simulink subsystem "DoubleActingPistonCylinderControlledValves"  (R2025b)
settings: Solver=VariableStepAuto  StartTime=0.0  StopTime=10.0  RelTol=1e-3
libraries: customization_lib x7, nesl_utility x2, fl_lib x1
settings Model: Creator=ndegoede  LastModifiedBy=ndegoede

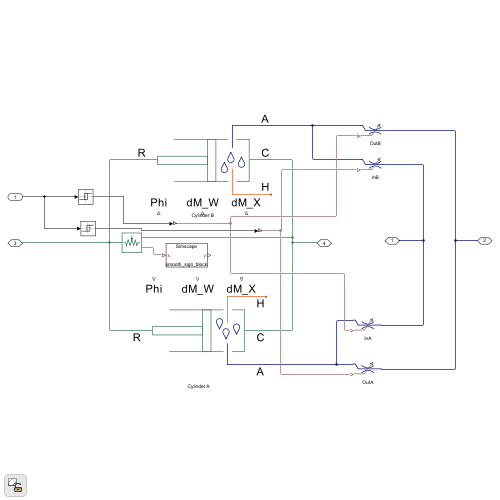
[thumbnail: Simulink's stored preview of the top-level diagram]
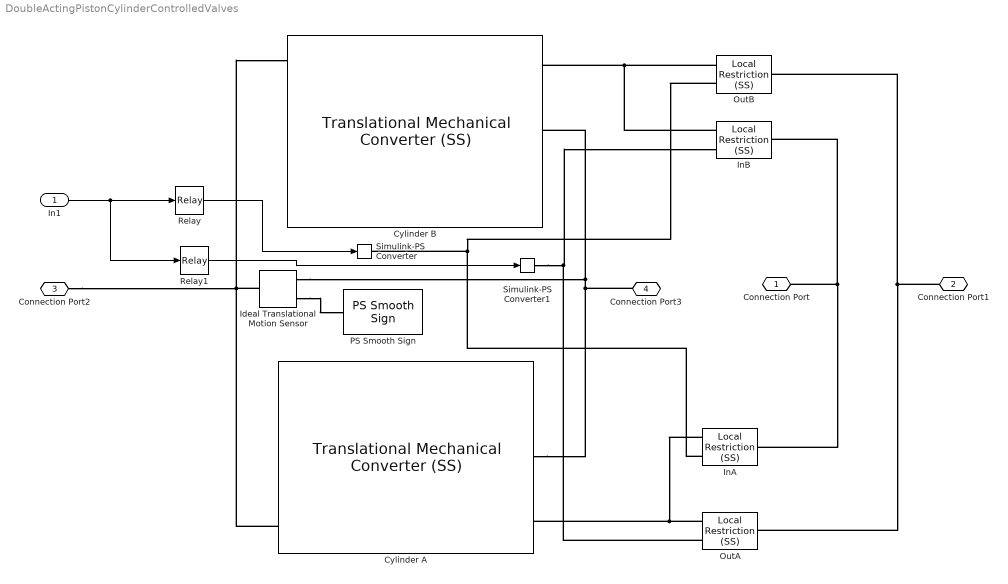
== system DoubleActingPistonCylinderControlledValves ==
  In1 : Inport
  Cylinder A : customization_lib/solution/elements/Translational Mechanical Converter (SS)  mech_orientation=foundation.enum.MechOrientationTranslational.Positive  length_init=7 m  interface_area=0.26 m^2  dead_volume=0.26*2 m^3  area_A=0.1 m^2  pressure_spec=foundation.enum.pressure_spec.atmospheric  environment_pressure=0.101325 MPa  m_measure=false  p_measure=false  t_measure=false  x_measure=false  dynamic_compressibility=false  p0=4 MPa  T0=293.15 K  p_nominal=0.101325 MPa  T_nominal=293.15 K  custom_ports=false  length_A=1e-3 m  x_I_specify=on  x_I_priority=High  x_I=36 kg/m^3  x_I_nominal_specify=off  x_I_nominal_value=1  x_I_nominal_unit=kg/m^3
      settings: SourceProductName=Customization  InternalSimscapePortConfiguration="{\"Bottom\":[{\"id\":\"dM_X\",\"label\":\"dM_X\",\"type\":\"input\"},{\"id\":\"dM_W\",\"label\":\"dM_W\",\"type\":\"input\"},{\"id\":\"Phi\",\"label\":\"Phi\",\"type\":\"input\"}],\"Left\":[{\"id\":\"A\",\"label\":\"A\",\"type\":\"customization.solution.solution\"},{\"id\":\"C\",\"label\":\"C\",\"type\":\"foundation.mechanical.translational.translational\"},{\"id\":\"H\",\"label\":\"H\",\"type\":\"foundation.thermal.thermal\"}],\"Right\":[{\"id\":\"R\",\"label\":\"R\",\"type\":\"foundation.mechanical.translational.translational\"}],\"Top\":[]}"
  "Cylinder B " : customization_lib/solution/elements/Translational Mechanical Converter (SS)  mech_orientation=foundation.enum.MechOrientationTranslational.Negative  length_init=-7 m  interface_area=0.26 m^2  dead_volume=2*0.26 m^3  area_A=0.1 m^2  pressure_spec=foundation.enum.pressure_spec.atmospheric  environment_pressure=0.101325 MPa  m_measure=false  p_measure=false  t_measure=false  x_measure=false  dynamic_compressibility=false  p0=4 MPa  T0=293.15 K  p_nominal=0.101325 MPa  T_nominal=293.15 K  custom_ports=false  length_A=1e-3 m  x_I_specify=on  x_I_priority=High  x_I=36 kg/m^3  x_I_nominal_specify=off  x_I_nominal_value=1  x_I_nominal_unit=kg/m^3
      settings: SourceProductName=Customization  InternalSimscapePortConfiguration="{\"Bottom\":[{\"id\":\"dM_X\",\"label\":\"dM_X\",\"type\":\"input\"},{\"id\":\"dM_W\",\"label\":\"dM_W\",\"type\":\"input\"},{\"id\":\"Phi\",\"label\":\"Phi\",\"type\":\"input\"}],\"Left\":[{\"id\":\"A\",\"label\":\"A\",\"type\":\"customization.solution.solution\"},{\"id\":\"C\",\"label\":\"C\",\"type\":\"foundation.mechanical.translational.translational\"},{\"id\":\"H\",\"label\":\"H\",\"type\":\"foundation.thermal.thermal\"}],\"Right\":[{\"id\":\"R\",\"label\":\"R\",\"type\":\"foundation.mechanical.translational.translational\"}],\"Top\":[]}"
  Ideal Translational Motion Sensor : fl_lib/Mechanical/Mechanical Sensors/Ideal Translational Motion Sensor  reference=foundation.enum.MeasurementReference.difference  acceleration_port=false  velocity_port=true  position_port=false  offset=0 m
      settings: InternalSimscapePortConfiguration="{\"Bottom\":[],\"Left\":[{\"id\":\"R\",\"label\":\"R\",\"type\":\"foundation.mechanical.translational.translational\"}],\"Right\":[{\"id\":\"C\",\"label\":\"C\",\"type\":\"foundation.mechanical.translational.translational\"},{\"id\":\"V\",\"label\":\"V\",\"type\":\"output\"}],\"Top\":[]}"
  InA : customization_lib/solution/elements/Local Restriction (SS)  restriction_type=foundation.enum.restriction_type.variable  restriction_area=0.001 m^2  min_area=1e-5 m^2  max_area=0.05 m^2  area=0.1 m^2  Cd=0.7  Re_c=150  pressure_recovery=simscape.enum.onoff.off  custom_ports=false  length_A=1e-3 m  length_B=1e-3 m
      settings: SourceProductName=Customization  InternalSimscapePortConfiguration="{\"Bottom\":[],\"Left\":[{\"id\":\"A\",\"label\":\"A\",\"type\":\"customization.solution.solution\"},{\"id\":\"area_in\",\"label\":\"AR\",\"type\":\"input\"}],\"Right\":[{\"id\":\"B\",\"label\":\"B\",\"type\":\"customization.solution.solution\"}],\"Top\":[]}"
  InB : customization_lib/solution/elements/Local Restriction (SS)  restriction_type=foundation.enum.restriction_type.variable  restriction_area=0.001 m^2  min_area=1e-5 m^2  max_area=0.05 m^2  area=0.1 m^2  Cd=0.7  Re_c=150  pressure_recovery=simscape.enum.onoff.off  custom_ports=false  length_A=1e-3 m  length_B=1e-3 m
      settings: SourceProductName=Customization  InternalSimscapePortConfiguration="{\"Bottom\":[],\"Left\":[{\"id\":\"A\",\"label\":\"A\",\"type\":\"customization.solution.solution\"},{\"id\":\"area_in\",\"label\":\"AR\",\"type\":\"input\"}],\"Right\":[{\"id\":\"B\",\"label\":\"B\",\"type\":\"customization.solution.solution\"}],\"Top\":[]}"
  OutA : customization_lib/solution/elements/Local Restriction (SS)  restriction_type=foundation.enum.restriction_type.variable  restriction_area=0.001 m^2  min_area=1e-5 m^2  max_area=0.05 m^2  area=0.1 m^2  Cd=0.7  Re_c=150  pressure_recovery=simscape.enum.onoff.on  custom_ports=false  length_A=1e-3 m  length_B=1e-3 m
      settings: SourceProductName=Customization  InternalSimscapePortConfiguration="{\"Bottom\":[],\"Left\":[{\"id\":\"A\",\"label\":\"A\",\"type\":\"customization.solution.solution\"},{\"id\":\"area_in\",\"label\":\"AR\",\"type\":\"input\"}],\"Right\":[{\"id\":\"B\",\"label\":\"B\",\"type\":\"customization.solution.solution\"}],\"Top\":[]}"
  OutB : customization_lib/solution/elements/Local Restriction (SS)  restriction_type=foundation.enum.restriction_type.variable  restriction_area=0.001 m^2  min_area=1e-5 m^2  max_area=0.05 m^2  area=0.1 m^2  Cd=0.7  Re_c=150  pressure_recovery=simscape.enum.onoff.off  custom_ports=false  length_A=1e-3 m  length_B=1e-3 m
      settings: SourceProductName=Customization  InternalSimscapePortConfiguration="{\"Bottom\":[],\"Left\":[{\"id\":\"A\",\"label\":\"A\",\"type\":\"customization.solution.solution\"},{\"id\":\"area_in\",\"label\":\"AR\",\"type\":\"input\"}],\"Right\":[{\"id\":\"B\",\"label\":\"B\",\"type\":\"customization.solution.solution\"}],\"Top\":[]}"
  PS Smooth Sign : customization_lib/function/PS Smooth Sign  x_th=1e-2
      settings: SourceProductName=Customization  InternalSimscapePortConfiguration="{\"Bottom\":[],\"Left\":[{\"id\":\"x\",\"label\":\"x\",\"type\":\"input\"}],\"Right\":[{\"id\":\"y\",\"label\":\"y\",\"type\":\"output\"}],\"Top\":[]}"
  Relay : Relay  OnSwitchValue=-0.05  OffSwitchValue=-0.05  OffOutputValue=-1
  Relay1 : Relay  OnSwitchValue=0.05  OffSwitchValue=0.05  OnOutputValue=-1  OffOutputValue=1
  Simulink-PS Converter : nesl_utility/Simulink-PS Converter  PhysicalDomain=network_engine_domain  SubClassName=ps_input  LeftPortType=input  RightPortType=output  PseudoPeriodic=off  Frequencies=[]  NoiseDistribution=none  NoiseParameters=[]  Unit=1  AffineConversion=off  FilteringAndDerivatives=zero  SimscapeFilterOrder=1  InputFilterTimeConstant=0.001  UdotUserProvided=0
  Simulink-PS Converter1 : nesl_utility/Simulink-PS Converter  PhysicalDomain=network_engine_domain  SubClassName=ps_input  LeftPortType=input  RightPortType=output  PseudoPeriodic=off  Frequencies=[]  NoiseDistribution=none  NoiseParameters=[]  Unit=1  AffineConversion=off  FilteringAndDerivatives=zero  SimscapeFilterOrder=1  InputFilterTimeConstant=0.001  UdotUserProvided=0
  Connection Port : PMIOPort  Side=Left
  Connection Port1 : PMIOPort  Port=2  Side=Left
  Connection Port2 : PMIOPort  Port=3  Side=Left
  Connection Port3 : PMIOPort  Port=4  Side=Left
  wires:
  Relay/1 -> Simulink-PS Converter/1
  In1/1 -> Relay/1, Relay1/1
  Relay1/1 -> Simulink-PS Converter1/1
  connections:
  OutB/LConn1 -- "Cylinder B "/LConn1 -- InB/LConn1
  OutB/RConn1 -- Connection Port1/RConn1 -- OutA/RConn1
  InB/RConn1 -- Connection Port/RConn1 -- InA/RConn1
  InA/LConn1 -- Cylinder A/LConn1 -- OutA/LConn1
  Ideal Translational Motion Sensor/LConn1 -- "Cylinder B "/RConn1 -- Cylinder A/RConn1 -- Connection Port2/RConn1
  "Cylinder B "/LConn2 -- Cylinder A/LConn2 -- Connection Port3/RConn1 -- Ideal Translational Motion Sensor/RConn1
  InA/LConn2 -- Simulink-PS Converter/RConn1 -- OutB/LConn2
  OutA/LConn2 -- Simulink-PS Converter1/RConn1 -- InB/LConn2
  Ideal Translational Motion Sensor/RConn2 -- PS Smooth Sign/LConn1
